simulink model "Projectile_1D_WithDrag"  (R2025b)
settings: Solver=VariableStepAuto  StartTime=0.0  StopTime=15  FixedStep=1e-2  MaxStep=1e-2  RelTol=1e-3
undefined symbols (not defined in the file): g
settings Model: Creator=esmithzb  LastModifiedBy=David
settings SolverCC: EnableFixedStepZeroCrossing=on

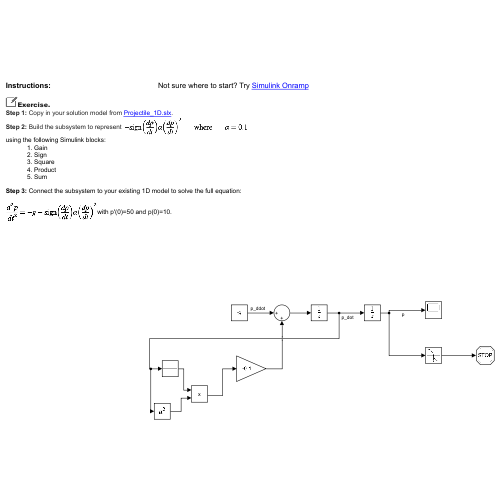
[thumbnail: Simulink's stored preview of the top-level diagram]
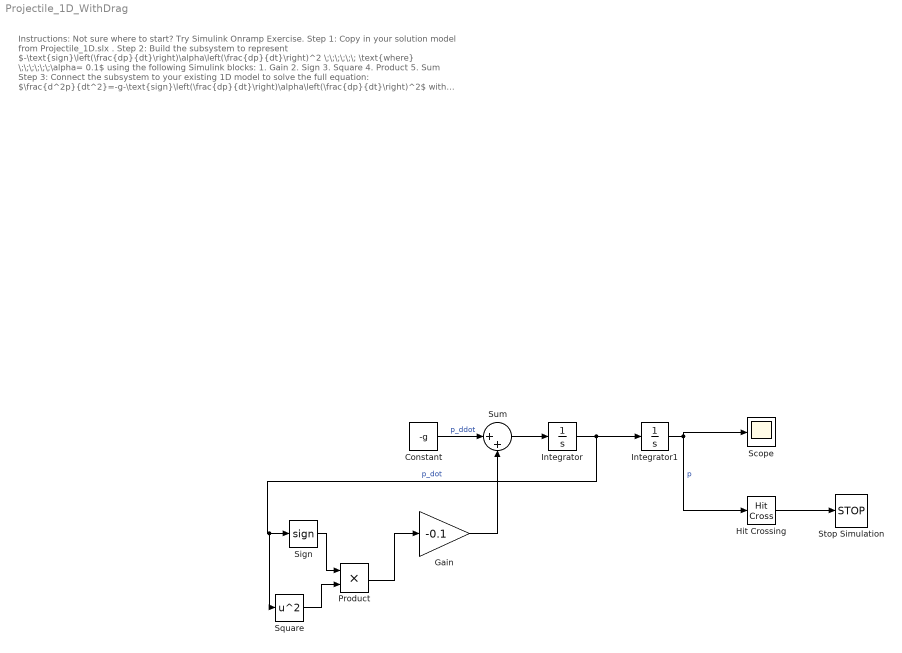
== system Projectile_1D_WithDrag ==
  note: Instructions: Not sure where to start? Try Simulink Onramp
      |
      | Exercise.
      | Step 1: Copy in your solution model from Projectile_1D.slx .
      | Step 2: Build the subsystem to represent $-\text{sign}\left(\frac{dp}{dt}\right)\alpha\left(\frac{dp}{dt}\right)^2 \;\;\;\;\;\; \text{where} \;\;\;\;\;\;\alpha= 0.1$
      | using the following Simulink blocks:
      | 1. Gain
      | 2. Sign
      | 3. Square
      | 4. Product
      | 5. Sum
      | Step 3: Connect the subsystem to your existing 1D model to solve the full equation: $\frac{d^2p}{dt^2}=-g-\text{sign}\left(\frac{dp}{dt}\right)\alpha\left(\frac{dp}{dt}\right)^2$ with p'(0)=50 and p(0)=10.
  Constant : Constant  Value=-g
  Gain : Gain  Gain=-0.1
  Hit Crossing : HitCross  HitCrossingDirection=falling
  Integrator : Integrator  InitialCondition=60
  Integrator1 : Integrator  InitialCondition=10
  Product : Product
  Scope : Scope
      settings: ActiveDisplayYMinimum=-3.397910804918713  ActiveDisplayYMaximum=31.653029473315893
  Sign : Signum
  Square : Math  Operator=square
  Stop Simulation : Stop
  Sum : Sum  Inputs=|++
  wires:
  Hit Crossing/1 -> Stop Simulation/1
  Integrator1/1 -> Scope/1, Hit Crossing/1  "p"
  Integrator/1 -> Square/1, Sign/1, Integrator1/1  "p_dot"
  Constant/1 -> Sum/1  "p_ddot"
  Sum/1 -> Integrator/1
  Sign/1 -> Product/1
  Square/1 -> Product/2
  Product/1 -> Gain/1
  Gain/1 -> Sum/2
